simulink model "Reformable_AI_2025"  (R2025b)
settings: Solver=ode23t  StartTime=0.0  StopTime=150  FixedStep=0.01  RelTol=1e-3
InitFcn:
  | load('PV_Params_Stage1.mat'); load('PV_Params_Stage2.mat');
values from neighbouring files (symbols this model uses):
  Iph_ref = P.Iph_ref*(1 - K.k_Iph*D)    [PaperFigures.m]
  n = lower(name)    [Stage10C_inventory.m]    (also in Stage10F2_make_manifest.m = size(rows,1); Stage10F_make_manifest.m = size(rows,1); Stage10F_run_one.m = 1; Stage10_assemble_dataset.m = height(T))
  OCV_tbl = [11.6 11.8 11.9 12.1 12.2 12.3 12.4 12.5 12.6 12.7 12.8]    [Battery_Param_Definition.m]
  Q = 7    [Battery_Param_Definition.m]
  q = 1.602176634e-19    [PaperFigures.m]    (also in Stage10C_inventory.m = L(strcmp({L.folder}, fl{k})); Stage10F2_make_manifest.m = M(M.regime == "A" & abs(M.bD - L) < 1e-12, :); Stage10F_make_manifest.m = M(M.regime == "A" & abs(M.bD - L) < 1e-12, :); Stage10G2_final_test.m = zeros(1, numel(seeds)))
  R0 = 0.03    [Battery_Param_Definition.m]    (also in PaperFigures.m = B.R0*(1 + KB.k_R0*D))
  R1 = 0.015    [Battery_Param_Definition.m]    (also in PaperFigures.m = B.R1*(1 + KB.k_R1*D))
  Rs = P.Rs*(1 + K.k_Rs*D)    [PaperFigures.m]
  Rsh = P.Rsh*(1 - K.k_Rsh*D)    [PaperFigures.m]
  SOC_bp = [0 10 20 30 40 50 60 70 80 90 100]    [Battery_Param_Definition.m]
  SOC_init = 100    [Battery_Param_Definition.m]
undefined symbols (not defined in the file or in its folder): Battery_Twin_C1, Battery_Twin_Capacity, Battery_Twin_OCV_tbl, Battery_Twin_R0, Battery_Twin_R1, Battery_Twin_SOC_bp, Battery_Twin_SOC_init, Battery_Twin_Vp_init, bias_G, bias_I_batt, bias_I_pv, bias_T_batt, bias_Tc, bias_V_batt, bias_V_pv, dG, dI_batt, dI_pv, drift_G, drift_I_batt, drift_I_pv, drift_T_batt, drift_Tc, drift_V_batt, drift_V_pv, dT_batt, dTc, dV_batt, dV_pv, Eg, ExcessiveNoise_Sigma, ExcessiveNoise_Sigma_batt, ExtraDrift_Rate, ExtraDrift_Rate_batt, FaultBias_Value, FaultBias_Value_batt, FaultSat_Max, FaultSat_Max_batt, FaultSat_Min, FaultSat_Min_batt, G_max, G_min, Gref, I0_ref, I_batt_max, I_batt_min, I_pv_max, I_pv_min, IntermittentDropoutProb, IntermittentDropoutProb_batt, Isc_ref, k_B, k_Iph, k_Q, k_R0, k_R1, k_Rs, k_Rsh, Ki, noise_G ... (+44)
libraries: fl_lib x7, nesl_utility x6
(part 1 of 3)
settings Model: Creator=inspiredkhalid  LastModifiedBy=inspiredkhalid
settings DataIOCC: InspectSignalLogs=on  LoggingToFile=on
settings SimscapeCC: SimscapeNominalValues="[{\"value\":\"1\",\"unit\":\"A\"},{\"value\":\"1\",\"unit\":\"bar\"},{\"value\":\"1\",\"unit\":\"cm^2\"},{\"value\":\"1\",\"unit\":\"cm^3/s\"},{\"value\":\"1\",\"unit\":\"kJ/kg\"},{\"value\":\"1\",\"unit\":\"kW\"},{\"value\":\"1\",\"unit\":\"l\"},{\"value\":\"1\",\"unit\":\"N\"},{\"value\":\"1\",\"unit\":\"N*m\"},{\"value\":\"1\",\"unit\":\"V\"},{\"value\":\"0.001\",\"unit\":\"Wb\"}]"  SimscapeLogType=all  SimscapeLogDataHistory=10000.0

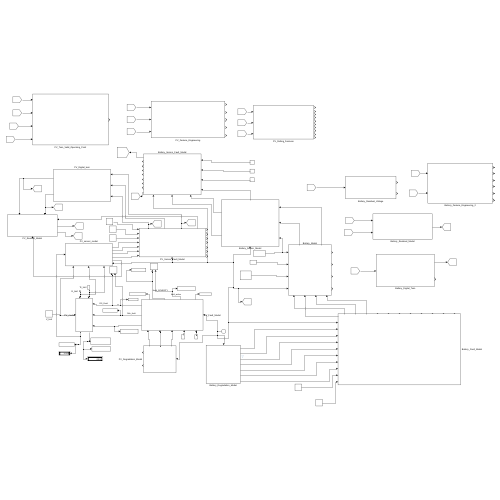
[thumbnail: Simulink's stored preview of the top-level diagram]
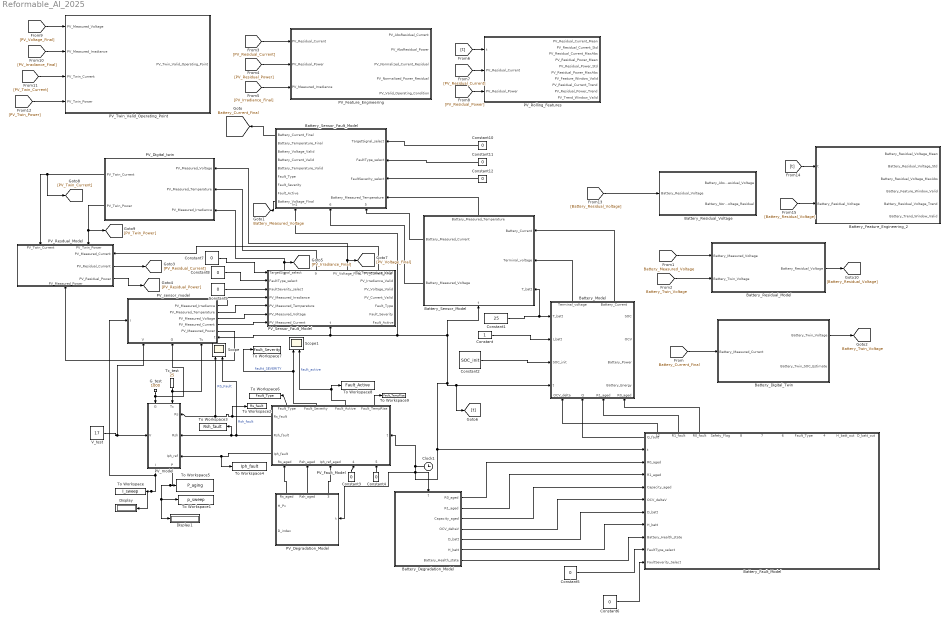
== system Reformable_AI_2025 ==
  Battery_Degradation_Model : Subsystem
      settings: PortSchema="{\"entries\":[{\"content\":{\"sides\":[{\"content\":{},\"type\":\"ConnectorPlacement.EquallySpacedRectSide\",\"uuid\":\"1b4fcb6b-66e9-48a9-b94c-f37550c0d7a8\"},{\"content\":{\"connectorIds\":[\"Out1\",\"Out2\",\"Out3\",\"Out4\",\"Out5\",\"Out6\",\"Out7\"],\"side\":\"RIGHT\"},\"type\":\"ConnectorPlacement.EquallySpacedRectSide\",\"uuid\":\"dcdb6d26-adba-4e3a-bfcc-7c50a5c7991f\"},{\"content\":{\"connectorIds\":[\"In1\"],\"side\":\"TOP\"},\"type\":\"ConnectorPlacement.EquallySpacedRectSide\",\"uuid\":\"b25d0552-795d-45d8-a626-a317e68fea8d\"}]},\"type\":\"ConnectorPlacement.EquallySpacedConnector\",\"uuid\":\"9e5bfc09-0161-4367-81be-9c2477d62c24\"}],\"packageUris\":[\"http://schema.mathworks.com/mf0/Connector/R2020b\"],\"version\":\"1.0\"}"
  Battery_Digital_Twin : Subsystem
  Battery_Fault_Model : Subsystem
      settings: PortSchema="{\"entries\":[{\"content\":{\"sides\":[{\"content\":{\"connectorIds\":[\"Out2\",\"Out3\",\"Out4\",\"Out5\",\"Out6\",\"Out7\",\"Out8\",\"Out9\",\"Out10\",\"Out11\",\"Out12\"]},\"type\":\"ConnectorPlacement.EquallySpacedRectSide\",\"uuid\":\"def34507-6478-4697-aeae-74e25b473746\"},{\"content\":{\"side\":\"RIGHT\"},\"type\":\"ConnectorPlacement.EquallySpacedRectSide\",\"uuid\":\"87bcd390-fe0e-4abd-8b9d-54c064a4bd6d\"},{\"content\":{\"side\":\"TOP\"},\"type\":\"ConnectorPlacement.EquallySpacedRectSide\",\"uuid\":\"8f6c8a66-988e-41f7-b815-fcd3c2d9d78f\"},{\"content\":{\"connectorIds\":[\"Out1\",\"In1\",\"In2\",\"In3\",\"In4\",\"In5\",\"In6\",\"In7\",\"In8\",\"In9\",\"In10\"],\"side\":\"BOTTOM\"},\"type\":\"ConnectorPlacement.EquallySpacedRectSide\",\"uuid\":\"924b8843-b89f-47e7-822a-230388281c89\"}]},\"type\":\"ConnectorPlacement.EquallySpacedConnector\",\"uuid\":\"c1b2d8db-a7be-4210-8e53-ee90bd01277c\"}],\"packageUris\":[\"http://schema.mathworks.com/mf0/Connector/R2020b\"],\"version\":\"1.0\"}"
  Battery_Feature_Engineering_2 : Subsystem
  Battery_Model : Subsystem
      settings: PortSchema="{\"entries\":[{\"content\":{\"sides\":[{\"content\":{\"connectorIds\":[\"In1\",\"In2\",\"In3\",\"In4\"]},\"type\":\"ConnectorPlacement.EquallySpacedRectSide\",\"uuid\":\"1f826f09-865b-4468-8a42-72e18ef3aa2b\"},{\"content\":{\"connectorIds\":[\"Out1\",\"Out2\",\"Out3\",\"Out4\"],\"side\":\"RIGHT\"},\"type\":\"ConnectorPlacement.EquallySpacedRectSide\",\"uuid\":\"5b9b4b60-a535-4dce-8159-4a5785c765d9\"},{\"content\":{\"connectorIds\":[\"Out5\",\"Out6\"],\"side\":\"TOP\"},\"type\":\"ConnectorPlacement.EquallySpacedRectSide\",\"uuid\":\"94076c55-be25-4bb0-90ef-93115b7bfd8f\"},{\"content\":{\"connectorIds\":[\"In5\",\"In6\",\"In7\",\"In8\"],\"side\":\"BOTTOM\"},\"type\":\"ConnectorPlacement.EquallySpacedRectSide\",\"uuid\":\"71d397e3-66ba-4153-89ad-3ec2a9926a6f\"}]},\"type\":\"ConnectorPlacement.EquallySpacedConnector\",\"uuid\":\"7a014506-dacd-4037-985d-2e24f4bfe43d\"}],\"packageUris\":[\"http://schema.mathworks.com/mf0/Connector/R2020b\"],\"version\":\"1.0\"}"
  Battery_Residual_Model : Subsystem
  Battery_Residual_Voltage : Subsystem
  Battery_Sensor_Fault_Model : Subsystem
      settings: PortSchema="{\"entries\":[{\"content\":{\"sides\":[{\"content\":{\"connectorIds\":[\"In1\",\"In2\",\"In3\",\"In4\"]},\"type\":\"ConnectorPlacement.EquallySpacedRectSide\",\"uuid\":\"bb3894e8-b902-4c6d-a9d1-c80b330f20fc\"},{\"content\":{\"connectorIds\":[\"Out1\",\"Out2\",\"Out3\",\"Out4\",\"Out5\",\"Out6\",\"Out7\",\"Out8\",\"Out9\"],\"side\":\"RIGHT\"},\"type\":\"ConnectorPlacement.EquallySpacedRectSide\",\"uuid\":\"10b9303a-ed2c-426d-b1e4-9725a6483ee8\"},{\"content\":{\"side\":\"TOP\"},\"type\":\"ConnectorPlacement.EquallySpacedRectSide\",\"uuid\":\"73c184b5-55b6-4d66-ad9e-4fe8ba237f9e\"},{\"content\":{\"connectorIds\":[\"In5\",\"In6\",\"In7\"],\"side\":\"BOTTOM\"},\"type\":\"ConnectorPlacement.EquallySpacedRectSide\",\"uuid\":\"5c55901c-dc1d-4ec5-aa71-af1f808363f4\"}]},\"type\":\"ConnectorPlacement.EquallySpacedConnector\",\"uuid\":\"e863a6e2-2521-4d2e-a149-f2fe745ce645\"}],\"packageUris\":[\"http://schema.mathworks.com/mf0/Connector/R2020b\"],\"version\":\"1.0\"}"
  Battery_Sensor_Model : Subsystem
      settings: PortSchema="{\"entries\":[{\"content\":{\"sides\":[{\"content\":{\"connectorIds\":[\"Out2\",\"Out3\"]},\"type\":\"ConnectorPlacement.EquallySpacedRectSide\",\"uuid\":\"8955ce44-6f38-48f5-9eff-64efe2779099\"},{\"content\":{\"connectorIds\":[\"In2\",\"In3\",\"In4\"],\"side\":\"RIGHT\"},\"type\":\"ConnectorPlacement.EquallySpacedRectSide\",\"uuid\":\"83e82735-d870-4b08-8880-ee704aeaa71f\"},{\"content\":{\"connectorIds\":[\"Out1\"],\"side\":\"TOP\"},\"type\":\"ConnectorPlacement.EquallySpacedRectSide\",\"uuid\":\"f0b9879b-0e80-439e-813e-88a693b75915\"},{\"content\":{\"connectorIds\":[\"In1\"],\"side\":\"BOTTOM\"},\"type\":\"ConnectorPlacement.EquallySpacedRectSide\",\"uuid\":\"7b7dd351-d288-44af-9c53-430aec26e948\"}]},\"type\":\"ConnectorPlacement.EquallySpacedConnector\",\"uuid\":\"dc77152e-fb82-4e41-8f3d-560bcd04aeca\"}],\"packageUris\":[\"http://schema.mathworks.com/mf0/Connector/R2020b\"],\"version\":\"1.0\"}"
  Clock1 : Clock
  Constant : Constant
  Constant1 : Constant  Value=25
  Constant{3..12} (10 alike) : Constant  Value=0
  Constant2 : Constant  Value=SOC_init
  Display : Display
  Display1 : Display
  G_test : Constant  Value=1000
  PV_Degradation_Model : Subsystem
      settings: PortSchema="{\"entries\":[{\"content\":{\"sides\":[{\"content\":{\"connectorIds\":[\"In1\"]},\"type\":\"ConnectorPlacement.EquallySpacedRectSide\",\"uuid\":\"fc7c08a7-a329-47c9-9fc8-bd6d0c7412cb\"},{\"content\":{\"connectorIds\":[\"Out1\",\"Out2\"],\"side\":\"RIGHT\"},\"type\":\"ConnectorPlacement.EquallySpacedRectSide\",\"uuid\":\"35a8a444-8a75-40e2-9eb4-ed34268f54da\"},{\"content\":{\"side\":\"TOP\"},\"type\":\"ConnectorPlacement.EquallySpacedRectSide\",\"uuid\":\"f1c409b4-d5ab-4e1c-b6d7-466c0f3dffa6\"},{\"content\":{\"connectorIds\":[\"Out3\",\"Out4\",\"Out5\"],\"side\":\"BOTTOM\"},\"type\":\"ConnectorPlacement.EquallySpacedRectSide\",\"uuid\":\"bca27c1f-7244-4b7d-89ff-49c1beb40a94\"}]},\"type\":\"ConnectorPlacement.EquallySpacedConnector\",\"uuid\":\"e415782b-02d5-4f08-91bd-00003c3592e4\"}],\"packageUris\":[\"http://schema.mathworks.com/mf0/Connector/R2020b\"],\"version\":\"1.0\"}"
  PV_Digital_twin : Subsystem
  PV_Fault_Model : Subsystem
      settings: PortSchema="{\"entries\":[{\"content\":{\"sides\":[{\"content\":{\"connectorIds\":[\"In1\",\"In2\",\"In3\",\"In4\",\"In5\"]},\"type\":\"ConnectorPlacement.EquallySpacedRectSide\",\"uuid\":\"8b731ac7-2216-400b-92c0-c5fd8078214b\"},{\"content\":{\"connectorIds\":[\"Out1\",\"Out2\",\"Out3\",\"Out4\"],\"side\":\"RIGHT\"},\"type\":\"ConnectorPlacement.EquallySpacedRectSide\",\"uuid\":\"014647c5-4381-4d16-b1c0-b8ab455ee411\"},{\"content\":{\"connectorIds\":[\"Out5\",\"Out6\",\"Out7\"],\"side\":\"TOP\"},\"type\":\"ConnectorPlacement.EquallySpacedRectSide\",\"uuid\":\"1f45222c-f229-4954-87dd-60ab673ad2f0\"},{\"content\":{\"connectorIds\":[\"In6\"],\"side\":\"BOTTOM\"},\"type\":\"ConnectorPlacement.EquallySpacedRectSide\",\"uuid\":\"4c4658ba-e21b-4f4c-8fc5-baa8c5c52617\"}]},\"type\":\"ConnectorPlacement.EquallySpacedConnector\",\"uuid\":\"427e782e-29c1-425f-8ec4-b06ea4eff844\"}],\"packageUris\":[\"http://schema.mathworks.com/mf0/Connector/R2020b\"],\"version\":\"1.0\"}"
  PV_Feature_Engineering : Subsystem
  PV_Resdual_Model : Subsystem
      settings: PortSchema="{\"entries\":[{\"content\":{\"sides\":[{\"content\":{},\"type\":\"ConnectorPlacement.EquallySpacedRectSide\",\"uuid\":\"b6a844ea-fc33-4046-8e41-66e00a162ef2\"},{\"content\":{\"connectorIds\":[\"In4\",\"Out1\",\"Out2\"],\"side\":\"RIGHT\"},\"type\":\"ConnectorPlacement.EquallySpacedRectSide\",\"uuid\":\"687d96a8-efea-420e-931b-35a130b52769\"},{\"content\":{\"connectorIds\":[\"In1\",\"In2\"],\"side\":\"TOP\"},\"type\":\"ConnectorPlacement.EquallySpacedRectSide\",\"uuid\":\"35b70589-b349-4394-ba77-bf30dc1caa8a\"},{\"content\":{\"connectorIds\":[\"In3\"],\"side\":\"BOTTOM\"},\"type\":\"ConnectorPlacement.EquallySpacedRectSide\",\"uuid\":\"b4c17054-bf3a-4618-abb5-cd6065b2fdb6\"}]},\"type\":\"ConnectorPlacement.EquallySpacedConnector\",\"uuid\":\"145bcfa6-69e9-4503-8576-d4854c5a5a59\"}],\"packageUris\":[\"http://schema.mathworks.com/mf0/Connector/R2020b\"],\"version\":\"1.0\"}"
  PV_Rolling_Features : Subsystem
  PV_Sensor_Fault_Model : Subsystem
      settings: PortSchema="{\"entries\":[{\"content\":{\"sides\":[{\"content\":{\"connectorIds\":[\"In1\",\"In2\",\"In3\",\"In4\",\"In5\",\"In6\",\"In7\"]},\"type\":\"ConnectorPlacement.EquallySpacedRectSide\",\"uuid\":\"1e67e2de-b259-436c-bcd9-e06714e4acbc\"},{\"content\":{\"connectorIds\":[\"Out1\",\"Out2\",\"Out3\",\"Out4\",\"Out5\",\"Out6\",\"Out7\"],\"side\":\"RIGHT\"},\"type\":\"ConnectorPlacement.EquallySpacedRectSide\",\"uuid\":\"fed75625-91c4-463a-8343-875db8c008fd\"},{\"content\":{\"connectorIds\":[\"Out8\",\"Out9\",\"Out10\",\"Out11\"],\"side\":\"TOP\"},\"type\":\"ConnectorPlacement.EquallySpacedRectSide\",\"uuid\":\"f60bd626-7f6d-4146-8351-a490a0f42c8a\"},{\"content\":{\"connectorIds\":[\"In8\"],\"side\":\"BOTTOM\"},\"type\":\"ConnectorPlacement.EquallySpacedRectSide\",\"uuid\":\"57953ecf-c9c3-41f5-9457-ff31205d2dee\"}]},\"type\":\"ConnectorPlacement.EquallySpacedConnector\",\"uuid\":\"e3cae6cc-0cb2-4c8c-ac91-b97a0780861c\"}],\"packageUris\":[\"http://schema.mathworks.com/mf0/Connector/R2020b\"],\"version\":\"1.0\"}"
  PV_Twin_Valid_Operating_Point : Subsystem
  PV_model : Subsystem
      settings: PortSchema="{\"entries\":[{\"content\":{\"sides\":[{\"content\":{\"connectorIds\":[\"In1\",\"In2\"]},\"type\":\"ConnectorPlacement.EquallySpacedRectSide\",\"uuid\":\"3a50d68a-8ea8-46a6-ad02-0f080f68b0a2\"},{\"content\":{\"connectorIds\":[\"Out1\",\"Out2\"],\"side\":\"RIGHT\"},\"type\":\"ConnectorPlacement.EquallySpacedRectSide\",\"uuid\":\"092f55fb-a7be-46a2-893e-2e9e60d96555\"},{\"content\":{\"connectorIds\":[\"In3\"],\"side\":\"TOP\"},\"type\":\"ConnectorPlacement.EquallySpacedRectSide\",\"uuid\":\"534c064b-53d0-494f-944d-ecbd004cd8da\"},{\"content\":{\"connectorIds\":[\"In4\",\"In5\",\"In6\"],\"side\":\"BOTTOM\"},\"type\":\"ConnectorPlacement.EquallySpacedRectSide\",\"uuid\":\"de40e54c-deaf-413c-8d15-7026379b682f\"}]},\"type\":\"ConnectorPlacement.EquallySpacedConnector\",\"uuid\":\"802b508a-319f-45a0-8063-6948fcaaf732\"}],\"packageUris\":[\"http://schema.mathworks.com/mf0/Connector/R2020b\"],\"version\":\"1.0\"}"
  PV_sensor_model : Subsystem
      settings: PortSchema="{\"entries\":[{\"content\":{\"sides\":[{\"content\":{\"connectorIds\":[\"In1\"]},\"type\":\"ConnectorPlacement.EquallySpacedRectSide\",\"uuid\":\"a02d4cda-723c-439e-90d8-70ed040ea171\"},{\"content\":{\"connectorIds\":[\"Out1\",\"Out2\",\"Out3\",\"Out4\",\"Out5\",\"In5\"],\"side\":\"RIGHT\"},\"type\":\"ConnectorPlacement.EquallySpacedRectSide\",\"uuid\":\"4d593adb-f3b3-43f8-9aef-6ad608411d44\"},{\"content\":{\"side\":\"TOP\"},\"type\":\"ConnectorPlacement.EquallySpacedRectSide\",\"uuid\":\"d32e8d54-74cc-4da5-8c08-e8fc23fa31c9\"},{\"content\":{\"connectorIds\":[\"In2\",\"In3\",\"In4\"],\"side\":\"BOTTOM\"},\"type\":\"ConnectorPlacement.EquallySpacedRectSide\",\"uuid\":\"081c40b8-ce17-4559-ae2b-235227de8849\"}]},\"type\":\"ConnectorPlacement.EquallySpacedConnector\",\"uuid\":\"0975a21e-08eb-4b13-8864-c9156be24474\"}],\"packageUris\":[\"http://schema.mathworks.com/mf0/Connector/R2020b\"],\"version\":\"1.0\"}"
  Scope : Scope  NumInputPorts=2
      settings: ActiveDisplayYMinimum=-1  ActiveDisplayYMaximum=1  DataLoggingVariableName=ScopeData3
  Scope1 : Scope  NumInputPorts=2
      settings: DataLoggingVariableName=ScopeData4
  Tc_test : Constant  Value=25
  To Workspace : ToWorkspace  VariableName=I_sweep  SaveFormat=Timeseries  SampleTime=-1
  To Workspace1 : ToWorkspace  VariableName=p_sweep  SaveFormat=Timeseries  SampleTime=-1
  To Workspace2 : ToWorkspace  VariableName=Rs_fault  SaveFormat=Timeseries  SampleTime=-1
  To Workspace3 : ToWorkspace  VariableName=Rsh_fault  SaveFormat=Timeseries  SampleTime=-1
  To Workspace4 : ToWorkspace  VariableName=Iph_fault  SaveFormat=Timeseries  SampleTime=-1
  To Workspace5 : ToWorkspace  VariableName=P_aging  SaveFormat=Timeseries  SampleTime=-1
  To Workspace6 : ToWorkspace  VariableName=Fault_Type  SaveFormat=Timeseries  SampleTime=-1
  To Workspace7 : ToWorkspace  VariableName=Fault_Severity  SaveFormat=Timeseries  SampleTime=-1
  To Workspace8 : ToWorkspace  VariableName=Fault_Active  SaveFormat=Timeseries  SampleTime=-1
  To Workspace9 : ToWorkspace  VariableName=Fault_TempRise  SaveFormat=Timeseries  SampleTime=-1
  V_test : Constant  Value=17
  tag scope: Battery_Current_Final=global, Battery_Measured_Voltage=global, Battery_Twin_Voltage=global
  wires:
  G_test/1 -> PV_sensor_model/3(G), PV_model/1(G)
  Tc_test/1 -> PV_sensor_model/4(Tc), PV_model/2(Tc)
  V_test/1 -> PV_sensor_model/2(V), PV_model/3(V)
  PV_Degradation_Model/5(Rs_aged) -> PV_Fault_Model/1(Rs_aged)
  PV_Degradation_Model/4(Rsh_aged) -> PV_Fault_Model/2(Rsh_aged)
  PV_Degradation_Model/3(Iph_ref_aged) -> PV_Fault_Model/3(Iph_ref_aged)
  Battery_Degradation_Model/1(R0_aged) -> Battery_Fault_Model/2(R0_aged)
  Battery_Degradation_Model/2(R1_aged) -> Battery_Fault_Model/3(R1_aged)
  Battery_Degradation_Model/3(Capacity_aged) -> Battery_Fault_Model/4(Capacity_aged)
  Battery_Degradation_Model/4(OCV_deltaV) -> Battery_Fault_Model/5(OCV_deltaV)
  PV_model/1(I) -> PV_sensor_model/1(I), Display/1, To Workspace/1
  Constant3/1 -> PV_Fault_Model/4(FaultType_select)
  Constant4/1 -> PV_Fault_Model/5(FaultSeverity_select)
  PV_Fault_Model/7(Rs_fault) -> To Workspace2/1, PV_model/4(Rs), Scope/1  "RS_Fault"
  PV_Fault_Model/6(Rsh_fault) -> PV_model/5(Rsh), To Workspace3/1, Scope/2  "Rsh_fault"
  PV_Fault_Model/5(Iph_fault) -> To Workspace4/1, PV_model/6(Iph_ref)
  PV_model/2(P) -> Display1/1, To Workspace1/1, To Workspace5/1
  PV_Fault_Model/2(Fault_Severity) -> Scope1/1, To Workspace7/1  "faultt_SEVERITY"
  PV_Fault_Model/3(Fault_Active) -> Scope1/2, To Workspace8/1  "fault_active"
  PV_Fault_Model/1(Fault_Type) -> To Workspace6/1
  PV_Fault_Model/4(Fault_TempRise) -> To Workspace9/1
  Constant1/1 -> Battery_Sensor_Model/4(T_batt), Battery_Model/1(T_batt)
  Constant2/1 -> Battery_Model/3(SOC_init)
  Constant/1 -> Battery_Model/2(I_batt)
  Battery_Degradation_Model/5(D_batt) -> Battery_Fault_Model/6(D_batt)
  Battery_Degradation_Model/6(H_batt) -> Battery_Fault_Model/7(H_batt)
  Battery_Degradation_Model/7(Battery_Health_state) -> Battery_Fault_Model/8(Battery_Health_state)
  Constant5/1 -> Battery_Fault_Model/9(FaultType_select)
  Constant6/1 -> Battery_Fault_Model/10(FaultSeverity_Select)
  Battery_Fault_Model/10(R0_fault) -> Battery_Model/8(R0_aged)
  Battery_Fault_Model/11(R1_fault) -> Battery_Model/7(R1_aged)
  Battery_Fault_Model/1(Q_fault) -> Battery_Model/6(Q)
  Battery_Fault_Model/12(OCV_delta_fault) -> Battery_Model/5(OCV_delta)
  PV_sensor_model/2(PV_Measured_Temperature) -> PV_Sensor_Fault_Model/5(PV_Measured_Temperature)
  PV_sensor_model/1(PV_Measured_Irradiance) -> PV_Sensor_Fault_Model/4(PV_Measured_Irradiance)
  PV_sensor_model/3(PV_Measured_Voltage) -> PV_Sensor_Fault_Model/6(PV_Measured_Voltage)
  PV_sensor_model/4(PV_Measured_Current) -> PV_Sensor_Fault_Model/7(PV_Measured_Current)
  Constant7/1 -> PV_Sensor_Fault_Model/1(TargetSignal_select)
  Constant8/1 -> PV_Sensor_Fault_Model/2(FaultType_select)
  Constant9/1 -> PV_Sensor_Fault_Model/3(FaultSeverity_select)
  Battery_Model/5(Terminal_voltage) -> Battery_Sensor_Model/3(Terminal_voltage)
  Battery_Model/6(Battery_Current) -> Battery_Sensor_Model/2(Battery_Current)
  Battery_Sensor_Model/3(Battery_Measured_Voltage) -> Battery_Sensor_Fault_Model/6(Battery_Measured_Voltage)
  Battery_Sensor_Model/2(Battery_Measured_Current) -> Battery_Sensor_Fault_Model/5(Battery_Measured_Current)
  Battery_Sensor_Model/1(Battery_Measured_Temperature) -> Battery_Sensor_Fault_Model/4(Battery_Measured_Temperature)
  Constant10/1 -> Battery_Sensor_Fault_Model/1(TargetSignal_select)
  Constant11/1 -> Battery_Sensor_Fault_Model/2(FaultType_select)
  Constant12/1 -> Battery_Sensor_Fault_Model/3(FaultSeverity_select)
  PV_Sensor_Fault_Model/9(PV_Temperature_Final) -> PV_Digital_twin/2(PV_Measured_Temperature)
  PV_Sensor_Fault_Model/10(PV_Voltage_Final) -> [PV_Voltage_Final], PV_Digital_twin/1(PV_Measured_Voltage)
  PV_Digital_twin/1(PV_Twin_Current) -> [PV_Twin_Current], PV_Resdual_Model/1(PV_Twin_Current)
  PV_sensor_model/5(PV_Measured_Power) -> PV_Resdual_Model/3(PV_Measured_Power)
  PV_Sensor_Fault_Model/11(PV_Current_Final) -> PV_Resdual_Model/4(PV_Measured_Current)
  Battery_Sensor_Fault_Model/1(Battery_Current_Final) -> [Battery_Current_Final]
  [Battery_Current_Final] -> Battery_Digital_Twin/1(Battery_Measured_Current)
  Battery_Sensor_Fault_Model/9(Battery_Voltage_FInal) -> [Battery_Measured_Voltage]
  [Battery_Measured_Voltage] -> Battery_Residual_Model/1(Battery_Measured_Voltage)
  Battery_Digital_Twin/1(Battery_Twin_Voltage) -> [Battery_Twin_Voltage]
  [Battery_Twin_Voltage] -> Battery_Residual_Model/2(Battery_Twin_Voltage)
  PV_Resdual_Model/1(PV_Residual_Current) -> [PV_Residual_Current]
  PV_Resdual_Model/2(PV_Residual_Power) -> [PV_Residual_Power]
  [PV_Residual_Current] -> PV_Feature_Engineering/1(PV_Residual_Current)
  [PV_Residual_Power] -> PV_Feature_Engineering/2(PV_Residual_Power)
  PV_Sensor_Fault_Model/8(PV_Irradiance_Final) -> [PV_Irradiance_Final], PV_Digital_twin/3(PV_Measured_Irradiance)
  [PV_Irradiance_Final] -> PV_Feature_Engineering/3(PV_Measured_Irradiance)
  Clock1/1 -> PV_sensor_model/5(t), PV_Sensor_Fault_Model/8(t), Battery_Sensor_Fault_Model/7(In1), Battery_Sensor_Model/1(t), [t], Battery_Model/4(t), Battery_Fault_Model/1(t), Battery_Degradation_Model/1(t), PV_Degradation_Model/1(t), PV_Fault_Model/6(t)
  [t] -> PV_Rolling_Features/1(t)
  [PV_Residual_Current] -> PV_Rolling_Features/2(PV_Residual_Current)
  [PV_Residual_Power] -> PV_Rolling_Features/3(PV_Residual_Power)
  [PV_Voltage_Final] -> PV_Twin_Valid_Operating_Point/1(PV_Measured_Voltage)
  [PV_Irradiance_Final] -> PV_Twin_Valid_Operating_Point/2(PV_Measured_Irradiance)
  PV_Digital_twin/2(PV_Twin_Power) -> [PV_Twin_Power], PV_Resdual_Model/2(PV_Twin_Power)
  [PV_Twin_Current] -> PV_Twin_Valid_Operating_Point/3(PV_Twin_Current)
  [PV_Twin_Power] -> PV_Twin_Valid_Operating_Point/4(PV_Twin_Power)
  Battery_Residual_Model/1(Battery_Residual_Voltage) -> [Battery_Residual_Voltage]
  [Battery_Residual_Voltage] -> Battery_Residual_Voltage/1(Battery_Residual_Voltage)
  [t] -> Battery_Feature_Engineering_2/1(t)
  [Battery_Residual_Voltage] -> Battery_Feature_Engineering_2/2(Battery_Residual_Voltage)

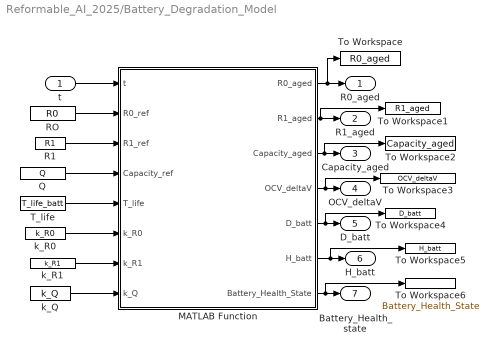
== system Reformable_AI_2025/Battery_Degradation_Model ==
  t : Inport
  MATLAB Function : MATLAB Function  TreatAsAtomicUnit=on
  Q : Constant  Value=Q
  R1 : Constant  Value=R1
  RO : Constant  Value=R0
  T_life : Constant  Value=T_life_batt
  To Workspace : ToWorkspace  VariableName=R0_aged  SaveFormat=Timeseries  SampleTime=-1
  To Workspace1 : ToWorkspace  VariableName=R1_aged  SaveFormat=Timeseries  SampleTime=-1
  To Workspace2 : ToWorkspace  VariableName=Capacity_aged  SaveFormat=Timeseries  SampleTime=-1
  To Workspace3 : ToWorkspace  VariableName=OCV_deltaV  SaveFormat=Timeseries  SampleTime=-1
  To Workspace4 : ToWorkspace  VariableName=D_batt  SaveFormat=Timeseries  SampleTime=-1
  To Workspace5 : ToWorkspace  VariableName=H_batt  SaveFormat=Timeseries  SampleTime=-1
  To Workspace6 : ToWorkspace  VariableName=Battery_Health_State  SaveFormat=Timeseries  SampleTime=-1
  k_Q : Constant  Value=k_Q
  k_R0 : Constant  Value=k_R0
  k_R1 : Constant  Value=k_R1
  R0_aged : Outport
  R1_aged : Outport  Port=2
  Capacity_aged : Outport  Port=3
  OCV_deltaV : Outport  Port=4
  D_batt : Outport  Port=5
  H_batt : Outport  Port=6
  Battery_Health_state : Outport  Port=7
  wires:
  t/1 -> MATLAB Function/1(t)
  RO/1 -> MATLAB Function/2(R0_ref)
  R1/1 -> MATLAB Function/3(R1_ref)
  Q/1 -> MATLAB Function/4(Capacity_ref)
  T_life/1 -> MATLAB Function/5(T_life)
  k_R0/1 -> MATLAB Function/6(k_R0)
  k_R1/1 -> MATLAB Function/7(k_R1)
  k_Q/1 -> MATLAB Function/8(k_Q)
  MATLAB Function/1(R0_aged) -> To Workspace/1, R0_aged/1
  MATLAB Function/2(R1_aged) -> To Workspace1/1, R1_aged/1
  MATLAB Function/3(Capacity_aged) -> To Workspace2/1, Capacity_aged/1
  MATLAB Function/4(OCV_deltaV) -> To Workspace3/1, OCV_deltaV/1
  MATLAB Function/5(D_batt) -> To Workspace4/1, D_batt/1
  MATLAB Function/6(H_batt) -> To Workspace5/1, H_batt/1
  MATLAB Function/7(Battery_Health_State) -> To Workspace6/1, Battery_Health_state/1

== system Reformable_AI_2025/Battery_Digital_Twin ==
  Battery_Measured_Current : Inport
  Constant : Constant  Value=Battery_Twin_Capacity
  Divide : Product  Inputs=*/
  Gain : Gain  Gain=-100/3600
  Integrator : Integrator  InitialCondition=Battery_Twin_SOC_init
  Integrator1 : Integrator  InitialCondition=Battery_Twin_Vp_init
  MATLAB Function : MATLAB Function  TreatAsAtomicUnit=on
  To Workspace : ToWorkspace  VariableName=Battery_Twin_Voltage  SaveFormat=Timeseries  SampleTime=-1
  To Workspace1 : ToWorkspace  VariableName=Battery_Twin_SOC_Estimate  SaveFormat=Timeseries  SampleTime=-1
  Battery_Twin_Voltage : Outport
  Battery_Twin_SOC_Estimate : Outport  Port=2
  wires:
  Battery_Measured_Current/1 -> MATLAB Function/1(Battery_Measured_Current), Gain/1
  MATLAB Function/1(Battery_Twin_Voltage) -> Battery_Twin_Voltage/1, To Workspace/1
  Gain/1 -> Divide/1
  Constant/1 -> Divide/2
  Divide/1 -> Integrator/1
  Integrator/1 -> Battery_Twin_SOC_Estimate/1, To Workspace1/1, MATLAB Function/2(Battery_Twin_SOC_Estimate)
  MATLAB Function/2(Battery_Twin_dVp_dt) -> Integrator1/1
  Integrator1/1 -> MATLAB Function/3(Battery_Twin_Vp)

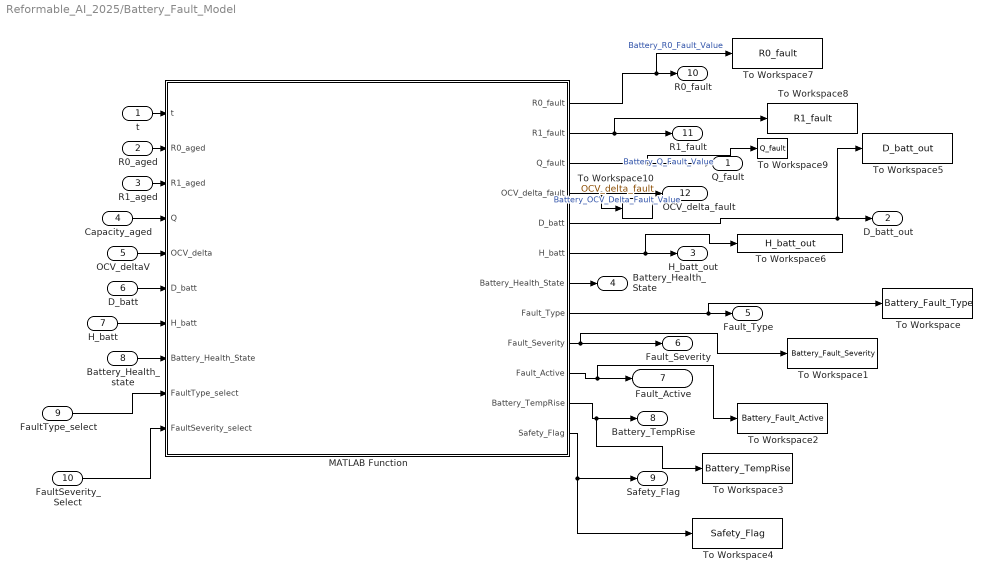
== system Reformable_AI_2025/Battery_Fault_Model ==
  t : Inport
  R0_aged : Inport  Port=2
  R1_aged : Inport  Port=3
  Capacity_aged : Inport  Port=4
  OCV_deltaV : Inport  Port=5
  D_batt : Inport  Port=6
  H_batt : Inport  Port=7
  Battery_Health_state : Inport  Port=8
  FaultType_select : Inport  Port=9
  FaultSeverity_Select : Inport  Port=10
  MATLAB Function : MATLAB Function  TreatAsAtomicUnit=on
  To Workspace : ToWorkspace  VariableName=Battery_Fault_Type  SaveFormat=Timeseries  SampleTime=-1
  To Workspace1 : ToWorkspace  VariableName=Battery_Fault_Severity  SaveFormat=Timeseries  SampleTime=-1
  To Workspace10 : ToWorkspace  VariableName=OCV_delta_fault  SaveFormat=Timeseries  SampleTime=-1
  To Workspace2 : ToWorkspace  VariableName=Battery_Fault_Active  SaveFormat=Timeseries  SampleTime=-1
  To Workspace3 : ToWorkspace  VariableName=Battery_TempRise  SaveFormat=Timeseries  SampleTime=-1
  To Workspace4 : ToWorkspace  VariableName=Safety_Flag  SaveFormat=Timeseries  SampleTime=-1
  To Workspace5 : ToWorkspace  VariableName=D_batt_out  SaveFormat=Timeseries  SampleTime=-1
  To Workspace6 : ToWorkspace  VariableName=H_batt_out  SaveFormat=Timeseries  SampleTime=-1
  To Workspace7 : ToWorkspace  VariableName=R0_fault  SaveFormat=Timeseries  SampleTime=-1
  To Workspace8 : ToWorkspace  VariableName=R1_fault  SaveFormat=Timeseries  SampleTime=-1
  To Workspace9 : ToWorkspace  VariableName=Q_fault  SaveFormat=Timeseries  SampleTime=-1
  Q_fault : Outport
  D_batt_out : Outport  Port=2
  H_batt_out : Outport  Port=3
  Battery_Health_State : Outport  Port=4
  Fault_Type : Outport  Port=5
  Fault_Severity : Outport  Port=6
  Fault_Active : Outport  Port=7
  Battery_TempRise : Outport  Port=8
  Safety_Flag : Outport  Port=9
  R0_fault : Outport  Port=10
  R1_fault : Outport  Port=11
  OCV_delta_fault : Outport  Port=12
  wires:
  t/1 -> MATLAB Function/1(t)
  R0_aged/1 -> MATLAB Function/2(R0_aged)
  R1_aged/1 -> MATLAB Function/3(R1_aged)
  Capacity_aged/1 -> MATLAB Function/4(Q)
  OCV_deltaV/1 -> MATLAB Function/5(OCV_delta)
  D_batt/1 -> MATLAB Function/6("D_batt ")
  H_batt/1 -> MATLAB Function/7("H_batt ")
  Battery_Health_state/1 -> MATLAB Function/8("Battery_Health_State ")
  FaultType_select/1 -> MATLAB Function/9(FaultType_select)
  FaultSeverity_Select/1 -> MATLAB Function/10(FaultSeverity_select)
  MATLAB Function/1(R0_fault) -> To Workspace7/1, R0_fault/1  "Battery_R0_Fault_Value"
  MATLAB Function/2(R1_fault) -> To Workspace8/1, R1_fault/1
  MATLAB Function/3(Q_fault) -> Q_fault/1, To Workspace9/1  "Battery_Q_Fault_Value"
  MATLAB Function/4(OCV_delta_fault) -> To Workspace10/1, OCV_delta_fault/1  "Battery_OCV_Delta_Fault_Value"
  MATLAB Function/6(H_batt) -> To Workspace6/1, H_batt_out/1
  MATLAB Function/5(D_batt) -> D_batt_out/1, To Workspace5/1
  MATLAB Function/7(Battery_Health_State) -> Battery_Health_State/1
  MATLAB Function/8(Fault_Type) -> To Workspace/1, Fault_Type/1
  MATLAB Function/9(Fault_Severity) -> To Workspace1/1, Fault_Severity/1
  MATLAB Function/10(Fault_Active) -> To Workspace2/1, Fault_Active/1
  MATLAB Function/11(Battery_TempRise) -> Battery_TempRise/1, To Workspace3/1
  MATLAB Function/12(Safety_Flag) -> To Workspace4/1, Safety_Flag/1

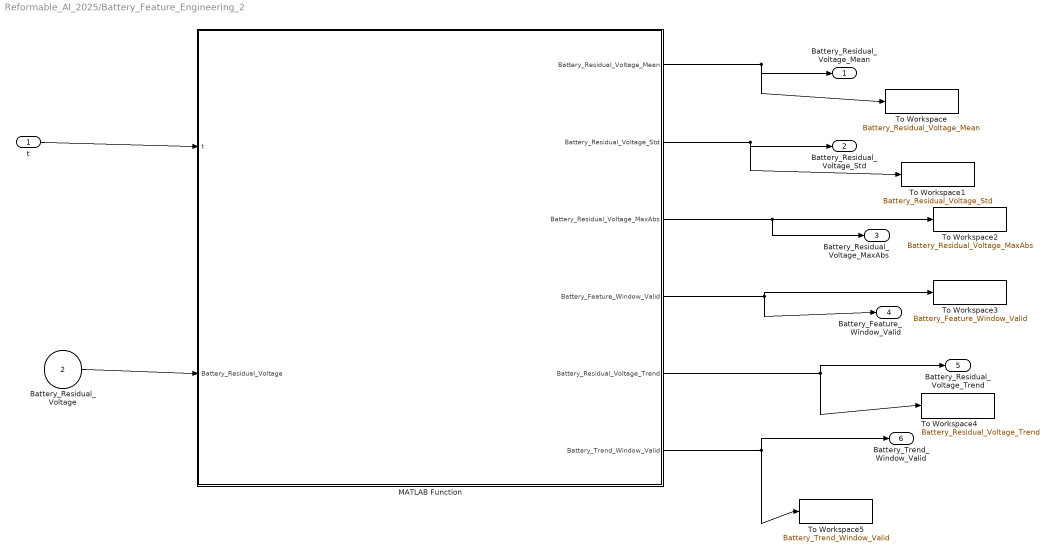
== system Reformable_AI_2025/Battery_Feature_Engineering_2 ==
  t : Inport
  Battery_Residual_Voltage : Inport  Port=2
  MATLAB Function : MATLAB Function  TreatAsAtomicUnit=on  SystemSampleTime=Stage9_Feature_SampleTime
  To Workspace : ToWorkspace  VariableName=Battery_Residual_Voltage_Mean  SaveFormat=Timeseries  SampleTime=-1
  To Workspace1 : ToWorkspace  VariableName=Battery_Residual_Voltage_Std  SaveFormat=Timeseries  SampleTime=-1
  To Workspace2 : ToWorkspace  VariableName=Battery_Residual_Voltage_MaxAbs  SaveFormat=Timeseries  SampleTime=-1
  To Workspace3 : ToWorkspace  VariableName=Battery_Feature_Window_Valid  SaveFormat=Timeseries  SampleTime=-1
  To Workspace4 : ToWorkspace  VariableName=Battery_Residual_Voltage_Trend  SaveFormat=Timeseries  SampleTime=-1
  To Workspace5 : ToWorkspace  VariableName=Battery_Trend_Window_Valid  SaveFormat=Timeseries  SampleTime=-1
  Battery_Residual_Voltage_Mean : Outport
  Battery_Residual_Voltage_Std : Outport  Port=2
  Battery_Residual_Voltage_MaxAbs : Outport  Port=3
  Battery_Feature_Window_Valid : Outport  Port=4
  Battery_Residual_Voltage_Trend : Outport  Port=5
  Battery_Trend_Window_Valid : Outport  Port=6
  wires:
  MATLAB Function/1(Battery_Residual_Voltage_Mean) -> To Workspace/1, Battery_Residual_Voltage_Mean/1
  MATLAB Function/2(Battery_Residual_Voltage_Std) -> To Workspace1/1, Battery_Residual_Voltage_Std/1
  MATLAB Function/3(Battery_Residual_Voltage_MaxAbs) -> Battery_Residual_Voltage_MaxAbs/1, To Workspace2/1
  MATLAB Function/4(Battery_Feature_Window_Valid) -> Battery_Feature_Window_Valid/1, To Workspace3/1
  t/1 -> MATLAB Function/1(t)
  Battery_Residual_Voltage/1 -> MATLAB Function/2(Battery_Residual_Voltage)
  MATLAB Function/5(Battery_Residual_Voltage_Trend) -> To Workspace4/1, Battery_Residual_Voltage_Trend/1
  MATLAB Function/6(Battery_Trend_Window_Valid) -> To Workspace5/1, Battery_Trend_Window_Valid/1

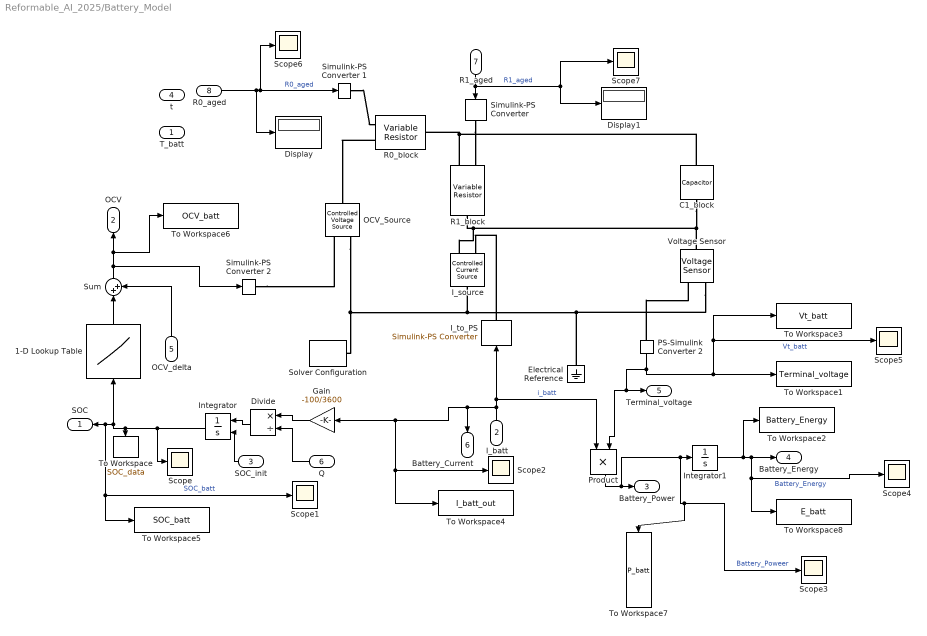
== system Reformable_AI_2025/Battery_Model ==
  T_batt : Inport
  I_batt : Inport  Port=2
  SOC_init : Inport  Port=3
  t : Inport  Port=4
  OCV_delta : Inport  Port=5
  Q : Inport  Port=6
  R1_aged : Inport  Port=7
  R0_aged : Inport  Port=8
  1-D Lookup Table : Lookup_n-D  NumberOfTableDimensions=1  BreakpointsForDimension1=SOC_bp  Table=OCV_tbl  InternalRulePriority=Speed  RndMeth=Simplest
  C1_block : fl_lib/Electrical/Electrical Elements/Capacitor  c=C1 F  r=1e-6 Ohm  g=0 1/Ohm  i_specify=off  i_priority=None  i=0 A  i_nominal_specify=off  i_nominal_value=1  i_nominal_unit=A  v_specify=off  v_priority=None  v=0 V  v_nominal_specify=off  v_nominal_value=1  v_nominal_unit=V  vc_specify=off  vc_priority=High  vc=0 V  vc_nominal_specify=off  vc_nominal_value=1  vc_nominal_unit=V
  Display : Display
  Display1 : Display
  Divide : Product  Inputs=*/
  Electrical Reference : fl_lib/Electrical/Electrical Elements/Electrical Reference
  Gain : Gain  Gain=-100/3600
  I_source : fl_lib/Electrical/Electrical Sources/Controlled Current Source
  I_to_PS : nesl_utility/Simulink-PS Converter  PhysicalDomain=network_engine_domain  SubClassName=ps_input  LeftPortType=input  RightPortType=output  PseudoPeriodic=off  Frequencies=[]  NoiseDistribution=none  NoiseParameters=[]  Unit=1  AffineConversion=off  FilteringAndDerivatives=provide  SimscapeFilterOrder=1  InputFilterTimeConstant=0.001  UdotUserProvided=0
  Integrator : Integrator  InitialConditionSource=external
  Integrator1 : Integrator
  OCV_Source : fl_lib/Electrical/Electrical Sources/Controlled Voltage Source
  PS-Simulink Converter 2 : nesl_utility/PS-Simulink Converter  PhysicalDomain=network_engine_domain  SubClassName=ps_output  LeftPortType=input  RightPortType=output  PseudoPeriodic=off  Frequencies=[]  VectorFormat=inherit  Unit=inherit  AffineConversion=off
  Product : Product
  R0_block : fl_lib/Electrical/Electrical Elements/Variable Resistor  Rmin=0 Ohm  thermalEnable=false  thermal_mass=1 J/K  i_specify=off  i_priority=None  i=0 A  i_nominal_specify=off  i_nominal_value=1  i_nominal_unit=A  v_specify=off  v_priority=None  v=0 V  v_nominal_specify=off  v_nominal_value=1  v_nominal_unit=V  T_specify=off  T_priority=None  T=300 K  T_nominal_specify=off  T_nominal_value=1  T_nominal_unit=K
  R1_block : fl_lib/Electrical/Electrical Elements/Variable Resistor  Rmin=0 Ohm  thermalEnable=false  thermal_mass=1 J/K  i_specify=off  i_priority=None  i=0 A  i_nominal_specify=off  i_nominal_value=1  i_nominal_unit=A  v_specify=off  v_priority=None  v=0 V  v_nominal_specify=off  v_nominal_value=1  v_nominal_unit=V  T_specify=off  T_priority=None  T=300 K  T_nominal_specify=off  T_nominal_value=1  T_nominal_unit=K
  Scope{,1..7} (8 alike) : Scope
      Scope2 settings: DataLoggingVariableName=ScopeData2
      Scope3 settings: DataLoggingVariableName=ScopeData5
      Scope4 settings: ActiveDisplayYMinimum=-1  ActiveDisplayYMaximum=1  DataLoggingVariableName=ScopeData6
      Scope5 settings: ActiveDisplayYMinimum=12.766194318471456  ActiveDisplayYMaximum=12.804241134423531  DataLoggingVariableName=ScopeData7
      Scope6 settings: ActiveDisplayYMinimum=-1  ActiveDisplayYMaximum=1  DataLoggingVariableName=ScopeData8
      Scope7 settings: ActiveDisplayYMinimum=-1  ActiveDisplayYMaximum=1  DataLoggingVariableName=ScopeData9
  "Simulink-PS Converter " : nesl_utility/Simulink-PS Converter  PhysicalDomain=network_engine_domain  SubClassName=ps_input  LeftPortType=input  RightPortType=output  PseudoPeriodic=off  Frequencies=[]  NoiseDistribution=none  NoiseParameters=[]  Unit=1  AffineConversion=off  FilteringAndDerivatives=provide  SimscapeFilterOrder=1  InputFilterTimeConstant=0.001  UdotUserProvided=0
  Simulink-PS Converter 1 : nesl_utility/Simulink-PS Converter  PhysicalDomain=network_engine_domain  SubClassName=ps_input  LeftPortType=input  RightPortType=output  PseudoPeriodic=off  Frequencies=[]  NoiseDistribution=none  NoiseParameters=[]  Unit=1  AffineConversion=off  FilteringAndDerivatives=provide  SimscapeFilterOrder=1  InputFilterTimeConstant=0.001  UdotUserProvided=0
  Simulink-PS Converter 2 : nesl_utility/Simulink-PS Converter  PhysicalDomain=network_engine_domain  SubClassName=ps_input  LeftPortType=input  RightPortType=output  PseudoPeriodic=off  Frequencies=[]  NoiseDistribution=none  NoiseParameters=[]  Unit=1  AffineConversion=off  FilteringAndDerivatives=provide  SimscapeFilterOrder=1  InputFilterTimeConstant=0.001  UdotUserProvided=0
  Solver Configuration : nesl_utility/Solver Configuration  PhysicalDomain=network_engine_domain  SubClassName=solver  LeftPortType=input  RightPortType=generic  Tones=[]  Harmonics=[]  SimulateNoise=off  Profile=off  UseLocalSampling=off  EnableSwitchedLinearOptims=on  FrequencyDomain=off  UseCCode=off  RelTol=0.001  AbsTol=0.001  MinStep=1e-09  ToWorkspace=off  RevertToSquareIcSolve=off  NumHomotopyIterations=100  PhasorMode=off  PhasorModeNumHarmonics=1  ConsistencySolver=NEWTON_XTOL_AFTER_FTOL  IndexReductionMethod=DerivativeReplacement  DoDC=off  ResidualTolerance=1e-09  ConsistencyTolSource=GLOBAL  ConsistencyAbsTol=0.001  ConsistencyRelTol=0.001  ConsistencyTolFactor=0.001  UseLocalSolver=off  LocalSolverChoice=NE_BACKWARD_EULER_ADVANCER  ResolveIndetEquations=on  FunctionEvalNumThread=1  LocalSolverSampleTime=0.001  DoFixedCost=off  MaxNonlinIter=3  MaxModeIter=2  ComputeImpulses=off  ImpulseIterations=2  LinearAlgebra=auto  LinearAlgebraNumThread=0  EquationFormulation=NE_TIME_EF  DelaysMemoryBudget=1024  AutomaticFiltering=on  FilteringTimeConstant=0.001  PartitionStorageMethod=AS_NEEDED  PartitionMemoryBudget=1024  PartitionMethod=ROBUST  MultibodyUseLocalSolver=off  MultibodyLocalSolverChoice=ODE1  MultibodyLocalSolverSampleTime=0.001
  Sum : Sum  Inputs=|++
  To Workspace : ToWorkspace  VariableName=SOC_data  SaveFormat=Timeseries  SampleTime=-1
  To Workspace1 : ToWorkspace  VariableName=Terminal_voltage  SaveFormat=Timeseries  SampleTime=-1
  To Workspace2 : ToWorkspace  VariableName=Battery_Energy  SaveFormat=Timeseries  SampleTime=-1
  To Workspace3 : ToWorkspace  VariableName=Vt_batt  SaveFormat=Timeseries  SampleTime=-1
  To Workspace4 : ToWorkspace  VariableName=I_batt_out  SaveFormat=Timeseries  SampleTime=-1
  To Workspace5 : ToWorkspace  VariableName=SOC_batt  SaveFormat=Timeseries  SampleTime=-1
  To Workspace6 : ToWorkspace  VariableName=OCV_batt  SaveFormat=Timeseries  SampleTime=-1
  To Workspace7 : ToWorkspace  VariableName=P_batt  SaveFormat=Timeseries  SampleTime=-1
  To Workspace8 : ToWorkspace  VariableName=E_batt  SaveFormat=Timeseries  SampleTime=-1
  "Voltage Sensor " : fl_lib/Electrical/Electrical Sensors/Voltage Sensor
  SOC : Outport
  OCV : Outport  Port=2
  Battery_Power : Outport  Port=3
  Battery_Energy : Outport  Port=4
  Terminal_voltage : Outport  Port=5
  Battery_Current : Outport  Port=6
  wires:
  R0_aged/1 -> Display/1, Scope6/1, Simulink-PS Converter 1/1  "R0_aged"
  R1_aged/1 -> Scope7/1, Display1/1, "Simulink-PS Converter "/1  "R1_aged"
  PS-Simulink Converter 2/1 -> Scope5/1, To Workspace3/1, To Workspace1/1, Product/2, Terminal_voltage/1  "Vt_batt"
  I_batt/1 -> Product/1, I_to_PS/1, To Workspace4/1, Scope2/1, Gain/1, Battery_Current/1  "i_batt"
  Gain/1 -> Divide/1
  Q/1 -> Divide/2
  Divide/1 -> Integrator/1
  Integrator/1 -> 1-D Lookup Table/1, Scope1/1, To Workspace5/1, SOC/1, To Workspace/1, Scope/1  "SOC_batt"
  Product/1 -> Scope3/1, To Workspace7/1, Integrator1/1, Battery_Power/1  "Battery_Poweer"
  Integrator1/1 -> To Workspace2/1, To Workspace8/1, Scope4/1, Battery_Energy/1  "Battery_Energy"
  SOC_init/1 -> Integrator/2
  1-D Lookup Table/1 -> Sum/1
  OCV_delta/1 -> Sum/2
  Sum/1 -> Simulink-PS Converter 2/1, OCV/1, To Workspace6/1
  connections:
  R0_block/LConn2 -- OCV_Source/LConn1
  C1_block/LConn1 -- R0_block/RConn1 -- R1_block/LConn2
  C1_block/RConn1 -- R1_block/RConn1 -- I_source/RConn2 -- "Voltage Sensor "/LConn1
  OCV_Source/RConn2 -- I_source/LConn1 -- "Voltage Sensor "/RConn2 -- Electrical Reference/LConn1 -- Solver Configuration/RConn1
  Simulink-PS Converter 1/RConn1 -- R0_block/LConn1
  "Simulink-PS Converter "/RConn1 -- R1_block/LConn1
  PS-Simulink Converter 2/LConn1 -- "Voltage Sensor "/RConn1
  I_to_PS/RConn1 -- I_source/RConn1
  Simulink-PS Converter 2/RConn1 -- OCV_Source/RConn1

== system Reformable_AI_2025/Battery_Residual_Model ==
  Battery_Measured_Voltage : Inport
  Battery_Twin_Voltage : Inport  Port=2
  MATLAB Function : MATLAB Function  TreatAsAtomicUnit=on
  To Workspace : ToWorkspace  VariableName=Battery_Residual_Voltage  SaveFormat=Timeseries  SampleTime=-1
  Battery_Residual_Voltage : Outport
  wires:
  Battery_Measured_Voltage/1 -> MATLAB Function/1(Battery_Measured_Voltage)
  Battery_Twin_Voltage/1 -> MATLAB Function/2(Battery_Twin_Voltage)
  MATLAB Function/1(Battery_Residual_Voltage) -> To Workspace/1, Battery_Residual_Voltage/1

== system Reformable_AI_2025/Battery_Residual_Voltage ==
  Battery_Residual_Voltage : Inport
  MATLAB Function : MATLAB Function  TreatAsAtomicUnit=on
  To Workspace : ToWorkspace  VariableName=Battery_Normalized_Voltage_Residual  SaveFormat=Timeseries  SampleTime=-1
  To Workspace1 : ToWorkspace  VariableName=Battery_AbsResidual_Voltage  SaveFormat=Timeseries  SampleTime=-1
  Battery_AbsResidual_Voltage : Outport
  Battery_Normalized_Voltage_Residual : Outport  Port=2
  wires:
  Battery_Residual_Voltage/1 -> MATLAB Function/1(Battery_Residual_Voltage)
  MATLAB Function/1(Battery_AbsResidual_Voltage) -> To Workspace1/1, Battery_AbsResidual_Voltage/1
  MATLAB Function/2(Battery_Normalized_Voltage_Residual) -> To Workspace/1, Battery_Normalized_Voltage_Residual/1

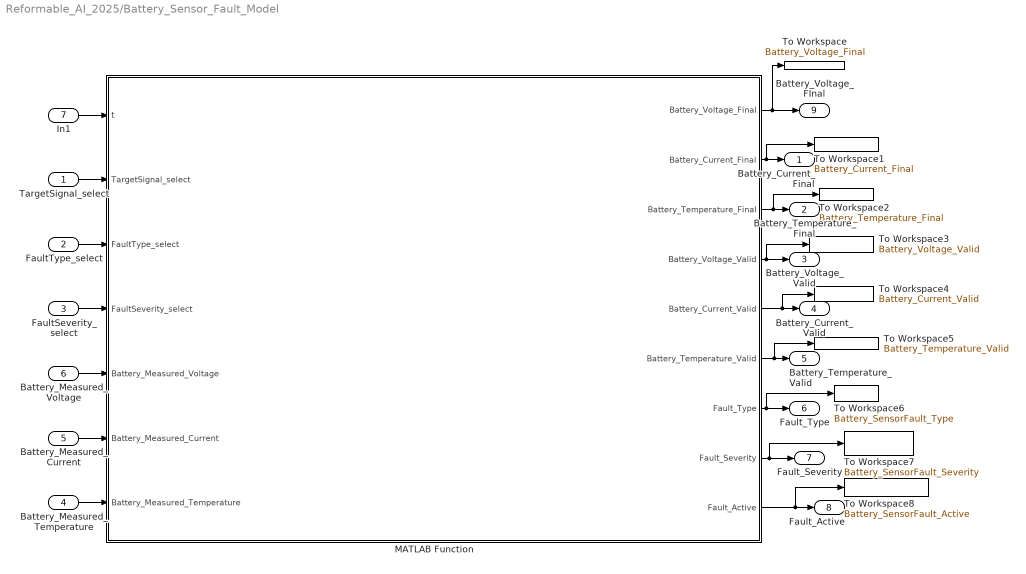
== system Reformable_AI_2025/Battery_Sensor_Fault_Model ==
  TargetSignal_select : Inport
  FaultType_select : Inport  Port=2
  FaultSeverity_select : Inport  Port=3
  Battery_Measured_Temperature : Inport  Port=4
  Battery_Measured_Current : Inport  Port=5
  Battery_Measured_Voltage : Inport  Port=6
  In1 : Inport  Port=7
  MATLAB Function : MATLAB Function  TreatAsAtomicUnit=on
  To Workspace : ToWorkspace  VariableName=Battery_Voltage_Final  SaveFormat=Timeseries  SampleTime=-1
  To Workspace1 : ToWorkspace  VariableName=Battery_Current_Final  SaveFormat=Timeseries  SampleTime=-1
  To Workspace2 : ToWorkspace  VariableName=Battery_Temperature_Final  SaveFormat=Timeseries  SampleTime=-1
  To Workspace3 : ToWorkspace  VariableName=Battery_Voltage_Valid  SaveFormat=Timeseries  SampleTime=-1
  To Workspace4 : ToWorkspace  VariableName=Battery_Current_Valid  SaveFormat=Timeseries  SampleTime=-1
  To Workspace5 : ToWorkspace  VariableName=Battery_Temperature_Valid  SaveFormat=Timeseries  SampleTime=-1
  To Workspace6 : ToWorkspace  VariableName=Battery_SensorFault_Type  SaveFormat=Timeseries  SampleTime=-1
  To Workspace7 : ToWorkspace  VariableName=Battery_SensorFault_Severity  SaveFormat=Timeseries  SampleTime=-1
  To Workspace8 : ToWorkspace  VariableName=Battery_SensorFault_Active  SaveFormat=Timeseries  SampleTime=-1
  Battery_Current_Final : Outport
  Battery_Temperature_Final : Outport  Port=2
  Battery_Voltage_Valid : Outport  Port=3
  Battery_Current_Valid : Outport  Port=4
  Battery_Temperature_Valid : Outport  Port=5
  Fault_Type : Outport  Port=6
  Fault_Severity : Outport  Port=7
  Fault_Active : Outport  Port=8
  Battery_Voltage_FInal : Outport  Port=9
  wires:
  In1/1 -> MATLAB Function/1(t)
  TargetSignal_select/1 -> MATLAB Function/2(TargetSignal_select)
  FaultType_select/1 -> MATLAB Function/3(FaultType_select)
  FaultSeverity_select/1 -> MATLAB Function/4(FaultSeverity_select)
  Battery_Measured_Voltage/1 -> MATLAB Function/5(Battery_Measured_Voltage)
  Battery_Measured_Current/1 -> MATLAB Function/6(Battery_Measured_Current)
  Battery_Measured_Temperature/1 -> MATLAB Function/7(Battery_Measured_Temperature)
  MATLAB Function/1(Battery_Voltage_Final) -> Battery_Voltage_FInal/1, To Workspace/1
  MATLAB Function/2(Battery_Current_Final) -> To Workspace1/1, Battery_Current_Final/1
  MATLAB Function/3(Battery_Temperature_Final) -> To Workspace2/1, Battery_Temperature_Final/1
  MATLAB Function/4(Battery_Voltage_Valid) -> To Workspace3/1, Battery_Voltage_Valid/1
  MATLAB Function/5(Battery_Current_Valid) -> To Workspace4/1, Battery_Current_Valid/1
  MATLAB Function/6(Battery_Temperature_Valid) -> To Workspace5/1, Battery_Temperature_Valid/1
  MATLAB Function/7(Fault_Type) -> To Workspace6/1, Fault_Type/1
  MATLAB Function/8(Fault_Severity) -> To Workspace7/1, Fault_Severity/1
  MATLAB Function/9(Fault_Active) -> To Workspace8/1, Fault_Active/1

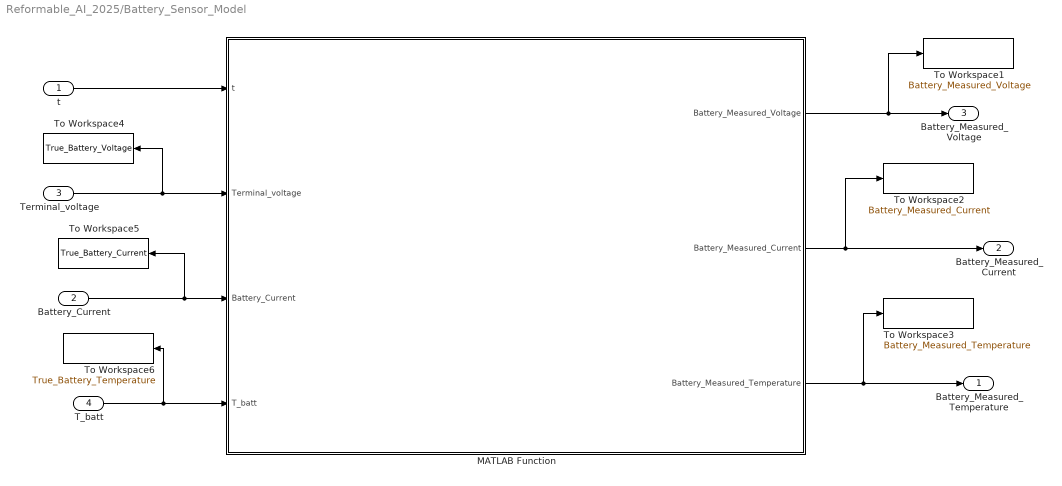
== system Reformable_AI_2025/Battery_Sensor_Model ==
  t : Inport
  Battery_Current : Inport  Port=2
  Terminal_voltage : Inport  Port=3
  T_batt : Inport  Port=4
  MATLAB Function : MATLAB Function  TreatAsAtomicUnit=on
  To Workspace1 : ToWorkspace  VariableName=Battery_Measured_Voltage  SaveFormat=Timeseries  SampleTime=-1
  To Workspace2 : ToWorkspace  VariableName=Battery_Measured_Current  SaveFormat=Timeseries  SampleTime=-1
  To Workspace3 : ToWorkspace  VariableName=Battery_Measured_Temperature  SaveFormat=Timeseries  SampleTime=-1
  To Workspace4 : ToWorkspace  VariableName=True_Battery_Voltage  SaveFormat=Timeseries  SampleTime=-1
  To Workspace5 : ToWorkspace  VariableName=True_Battery_Current  SaveFormat=Timeseries  SampleTime=-1
  To Workspace6 : ToWorkspace  VariableName=True_Battery_Temperature  SaveFormat=Timeseries  SampleTime=-1
  Battery_Measured_Temperature : Outport
  Battery_Measured_Current : Outport  Port=2
  Battery_Measured_Voltage : Outport  Port=3
  wires:
  T_batt/1 -> To Workspace6/1, MATLAB Function/4(T_batt)
  Battery_Current/1 -> To Workspace5/1, MATLAB Function/3(Battery_Current)
  Terminal_voltage/1 -> To Workspace4/1, MATLAB Function/2(Terminal_voltage)
  MATLAB Function/1(Battery_Measured_Voltage) -> To Workspace1/1, Battery_Measured_Voltage/1
  MATLAB Function/2(Battery_Measured_Current) -> To Workspace2/1, Battery_Measured_Current/1
  MATLAB Function/3(Battery_Measured_Temperature) -> To Workspace3/1, Battery_Measured_Temperature/1
  t/1 -> MATLAB Function/1(t)

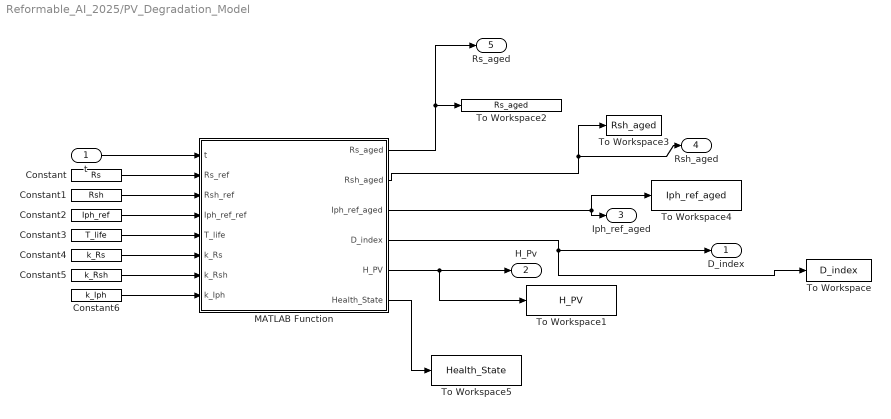
== system Reformable_AI_2025/PV_Degradation_Model ==
  t : Inport
  Constant : Constant  Value=Rs
  Constant1 : Constant  Value=Rsh
  Constant2 : Constant  Value=Iph_ref
  Constant3 : Constant  Value=T_life
  Constant4 : Constant  Value=k_Rs
  Constant5 : Constant  Value=k_Rsh
  Constant6 : Constant  Value=k_Iph
  MATLAB Function : MATLAB Function  TreatAsAtomicUnit=on
  To Workspace : ToWorkspace  VariableName=D_index  SaveFormat=Timeseries  SampleTime=-1
  To Workspace1 : ToWorkspace  VariableName=H_PV  SaveFormat=Timeseries  SampleTime=-1
  To Workspace2 : ToWorkspace  VariableName=Rs_aged  SaveFormat=Timeseries  SampleTime=-1
  To Workspace3 : ToWorkspace  VariableName=Rsh_aged  SaveFormat=Timeseries  SampleTime=-1
  To Workspace4 : ToWorkspace  VariableName=Iph_ref_aged  SaveFormat=Timeseries  SampleTime=-1
  To Workspace5 : ToWorkspace  VariableName=Health_State  SaveFormat=Timeseries  SampleTime=-1
  D_index : Outport
  H_Pv : Outport  Port=2
  Iph_ref_aged : Outport  Port=3
  Rsh_aged : Outport  Port=4
  Rs_aged : Outport  Port=5
  wires:
  t/1 -> MATLAB Function/1(t)
  Constant/1 -> MATLAB Function/2(Rs_ref)
  Constant1/1 -> MATLAB Function/3(Rsh_ref)
  Constant2/1 -> MATLAB Function/4(Iph_ref_ref)
  Constant3/1 -> MATLAB Function/5(T_life)
  Constant4/1 -> MATLAB Function/6(k_Rs)
  Constant5/1 -> MATLAB Function/7(k_Rsh)
  Constant6/1 -> MATLAB Function/8(k_Iph)
  MATLAB Function/2(Rsh_aged) -> To Workspace3/1, Rsh_aged/1
  MATLAB Function/3(Iph_ref_aged) -> Iph_ref_aged/1, To Workspace4/1
  MATLAB Function/4(D_index) -> To Workspace/1, D_index/1
  MATLAB Function/5(H_PV) -> To Workspace1/1, H_Pv/1
  MATLAB Function/1(Rs_aged) -> Rs_aged/1, To Workspace2/1
  MATLAB Function/6(Health_State) -> To Workspace5/1

== system Reformable_AI_2025/PV_Digital_twin ==
  PV_Measured_Voltage : Inport
  PV_Measured_Temperature : Inport  Port=2
  PV_Measured_Irradiance : Inport  Port=3
  MATLAB Function : MATLAB Function  TreatAsAtomicUnit=on
  To Workspace : ToWorkspace  VariableName=PV_Twin_Current  SaveFormat=Timeseries  SampleTime=-1
  To Workspace1 : ToWorkspace  VariableName=PV_Twin_Power  SaveFormat=Timeseries  SampleTime=-1
  PV_Twin_Current : Outport
  PV_Twin_Power : Outport  Port=2
  wires:
  PV_Measured_Irradiance/1 -> MATLAB Function/1(PV_Measured_Irradiance)
  PV_Measured_Temperature/1 -> MATLAB Function/2(PV_Measured_Temperature)
  PV_Measured_Voltage/1 -> MATLAB Function/3(PV_Measured_Voltage)
  MATLAB Function/1(PV_Twin_Current) -> To Workspace/1, PV_Twin_Current/1
  MATLAB Function/2(PV_Twin_Power) -> To Workspace1/1, PV_Twin_Power/1

== system Reformable_AI_2025/PV_Fault_Model ==
  Rs_aged : Inport
  Rsh_aged : Inport  Port=2
  Iph_ref_aged : Inport  Port=3
  FaultType_select : Inport  Port=4
  FaultSeverity_select : Inport  Port=5
  t : Inport  Port=6
  MATLAB Function : MATLAB Function  TreatAsAtomicUnit=on
  Fault_Type : Outport
  Fault_Severity : Outport  Port=2
  Fault_Active : Outport  Port=3
  Fault_TempRise : Outport  Port=4
  Iph_fault : Outport  Port=5
  Rsh_fault : Outport  Port=6
  Rs_fault : Outport  Port=7
  wires:
  FaultSeverity_select/1 -> MATLAB Function/6(FaultSeverity_select)
  FaultType_select/1 -> MATLAB Function/5(FaultType_select)
  Iph_ref_aged/1 -> MATLAB Function/4(Iph_ref_aged)
  Rsh_aged/1 -> MATLAB Function/3(Rsh_aged)
  Rs_aged/1 -> MATLAB Function/2(Rs_aged)
  t/1 -> MATLAB Function/1(t)
  MATLAB Function/1(Rs_fault) -> Rs_fault/1
  MATLAB Function/2(Rsh_fault) -> Rsh_fault/1
  MATLAB Function/3(Iph_fault) -> Iph_fault/1
  MATLAB Function/4(Fault_Type) -> Fault_Type/1
  MATLAB Function/5(Fault_Severity) -> Fault_Severity/1
  MATLAB Function/6(Fault_Active) -> Fault_Active/1
  MATLAB Function/7(Fault_TempRise) -> Fault_TempRise/1

== system Reformable_AI_2025/PV_Feature_Engineering ==
  PV_Residual_Current : Inport
  PV_Residual_Power : Inport  Port=2
  PV_Measured_Irradiance : Inport  Port=3
  MATLAB Function : MATLAB Function  TreatAsAtomicUnit=on
  To Workspace : ToWorkspace  VariableName=PV_Valid_Operating_Condition  SaveFormat=Timeseries  SampleTime=-1
  To Workspace1 : ToWorkspace  VariableName=PV_Normalized_Power_Residual  SaveFormat=Timeseries  SampleTime=-1
  To Workspace2 : ToWorkspace  VariableName=PV_Normalized_Current_Residual  SaveFormat=Timeseries  SampleTime=-1
  To Workspace3 : ToWorkspace  VariableName=PV_AbsResidual_Power  SaveFormat=Timeseries  SampleTime=-1
  To Workspace4 : ToWorkspace  VariableName=PV_AbsResidual_Current  SaveFormat=Timeseries  SampleTime=-1
  PV_AbsResidual_Current : Outport
  PV_AbsResidual_Power : Outport  Port=2
  PV_Normalized_Current_Residual : Outport  Port=3
  PV_Normalized_Power_Residual : Outport  Port=4
  PV_Valid_Operating_Condition : Outport  Port=5
  wires:
  PV_Residual_Current/1 -> MATLAB Function/1(PV_Residual_Current)
  PV_Residual_Power/1 -> MATLAB Function/2(PV_Residual_Power)
  PV_Measured_Irradiance/1 -> MATLAB Function/3(PV_Measured_Irradiance)
  MATLAB Function/1(PV_AbsResidual_Current) -> To Workspace4/1, PV_AbsResidual_Current/1
  MATLAB Function/2(PV_AbsResidual_Power) -> To Workspace3/1, PV_AbsResidual_Power/1
  MATLAB Function/3(PV_Normalized_Current_Residual) -> To Workspace2/1, PV_Normalized_Current_Residual/1
  MATLAB Function/4(PV_Normalized_Power_Residual) -> To Workspace1/1, PV_Normalized_Power_Residual/1
  MATLAB Function/5(PV_Valid_Operating_Condition) -> PV_Valid_Operating_Condition/1, To Workspace/1
